simulink model "coffee_machine_sim"  (R2025b)
settings: Solver=FixedStepDiscrete  StartTime=0.0  StopTime=12.0  FixedStep=0.01  RelTol=1e-3
settings Model: Creator=HP  LastModifiedBy=HP

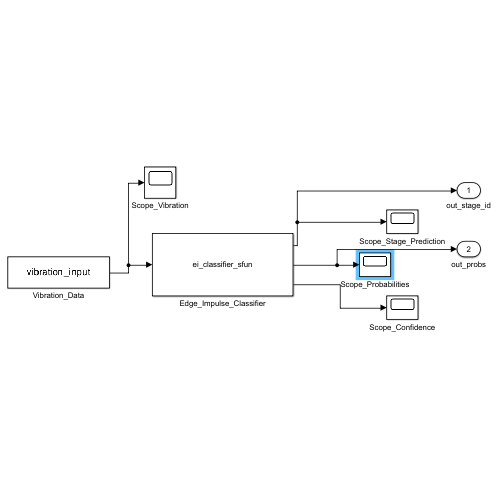
[thumbnail: Simulink's stored preview of the top-level diagram]
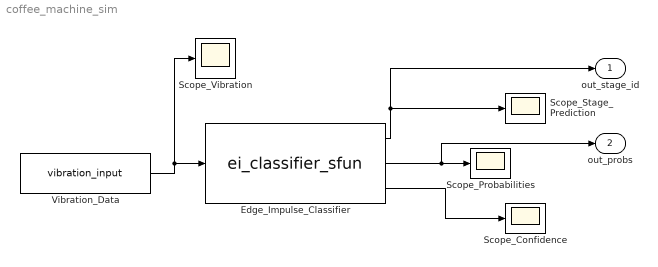
== system coffee_machine_sim ==
  Edge_Impulse_Classifier : S-Function  FunctionName=ei_classifier_sfun  Parameters=0.01, 10  SFunctionDeploymentMode=off  EnableBusSupport=off
  Scope_Confidence : Scope
      settings: ActiveDisplayYMinimum=0.349609375  ActiveDisplayYMaximum=1.072265625
  Scope_Probabilities : Scope
      settings: ActiveDisplayYMinimum=-0.12499999999999997  ActiveDisplayYMaximum=1.125
  Scope_Stage_Prediction : Scope
      settings: ActiveDisplayYMinimum=0.62500000000000011  ActiveDisplayYMaximum=4.375
  Scope_Vibration : Scope
      settings: ActiveDisplayYMinimum=-1.3713785891163157  ActiveDisplayYMaximum=12.213246301137566
  Vibration_Data : FromWorkspace  VariableName=vibration_input  SampleTime=0.01
  out_stage_id : Outport
  out_probs : Outport  Port=2
  wires:
  Vibration_Data/1 -> Scope_Vibration/1, Edge_Impulse_Classifier/1
  Edge_Impulse_Classifier/1 -> Scope_Stage_Prediction/1, out_stage_id/1
  Edge_Impulse_Classifier/2 -> out_probs/1, Scope_Probabilities/1
  Edge_Impulse_Classifier/3 -> Scope_Confidence/1
